simulink model "ASM_Traffic_new"  (R2024a)
settings: Solver=ode1  StartTime=SIM.tstart.v  StopTime=SIM.tend.v  FixedStep=SIM.StepSize.v  RelTol=1e-3
PostLoadFcn:
  | if any(exist('dsrtsu_mdlpostloadfcn', 'file') ~= 0), dsrtsu_mdlpostloadfcn('Execute', bdroot); end
  | try, asm_mdl_postloadfcn(bdroot, 'UpdateModel', 3600); catch, disp(lasterr); end,
InitFcn:
  | , if any(exist('rtifpga_mdlclblib', 'file') ~= 0), rtifpga_mdlclblib('Init', bdroot); end,
  | , if any(exist('dsmpb_private', 'file') ~= 0), dsmpb_private('dsmpb_mdlclblib', 'Init', bdroot); end,
undefined symbols (not defined in the file): _to_, a0b2, ASM_BrakeHydraulics_DemoSystems, ASM_VehicleDynamics_DemoSystems, b98103fe8ad365046cd0, BrakeCircuit, CPT, Crankshaft, DiscIntNeverNeededParam, dsmsi, FinalDriveAssembly, MDL, ModeSignals, Pos_BrakePedal_Maneuver, rad, RefSignals, s_to_rpm, SIM, SoftECU, Suspension, Tire, Transmission
libraries: ASM_Traffic_lib x135, simulink x100, ASM_Utils_lib x77, ASM_VehicleDynamics_lib x70, ASM_Environment_lib x22, dsmpblib x20, dsmsilib x15, MDLD_Utils_lib x10, ASM_BrakeHydraulics_lib x3
(part 18 of 63)

== system ASM_Traffic_new/DomainControl/DriverAssistance/Control/SoftECU_ACC ==
  UserInterface : Inport
  Interface_In : Inport  Port=2
  Bus Creator : BusCreator  Inputs=10
  Bus Selector1 : BusSelector  OutputSignals=SoftECU_ACC.Switches_ACC
  Bus Selector3 : BusSelector  OutputSignals=ExternalModel.v_x_Vehicle_CoG[km|h],ExternalModel.YawRate_Vehicle_CoG[deg|s],ExternalModel.Pos_FL_Wheel[x;y;z][m],ExternalModel.Pos_FR_Wheel[x;y;z][m],ExternalModel.r_Dyn_Tire[FL;FR;RL;RR][m],ExternalModel.Coef_RollingRes[FL;FR;RL;RR][],ExternalModel.Cw_x[],ExternalModel.i_FrontDrive[],ExternalModel.i_RearDrive[],ExternalModel.TrqDistri_Front_Rear[0_1][],ExternalModel.i_unsync_Trm[],ExternalModel.m_TotalVehicle[kg],ExternalModel.Trq_Fric_Engine[Nm],ExternalModel.Pos_AccPedal[%],ExternalModel.Pos_BrakePedal[%],ExternalModel.Slope_Veh_Road[%],ExternalModel.s_Vehicle_Road[m],ExternalModel.d_Vehicle_Road[m],ExternalModel.Dist_Fellows[m],ExternalModel.v_Rel_Fellows[m|s],ExternalModel.Angle_Hor_Rel_Fellows[deg],ExternalModel.s_Fellows_Ref[m],ExternalModel.d_Total_Fellows[m],ExternalModel.PosVec_MainPnt_Fellows[x;y;z][m],ExternalModel.Length_Fellows[m],ExternalModel.Width_Fellows[m],ExternalModel.Height_Fellows[m],ExternalModel.Object_ID[],ExternalModel.ECU_Commands[],ExternalModel.Reset[0|1]
  ModelDesk_MC_ID_SoftECU : ASM_Utils_lib/ModelDeskInterface/ModelDesk_MC  Tag=ASM_MAINCOMPONENT  Editable=off  MainComponent=SoftECU
  Soft_ECU_ACC : Subsystem
  ASMSignalBus : Outport  VectorParamsAs1DForOutWhenUnconnected=off
  Out : Outport  Port=2  VectorParamsAs1DForOutWhenUnconnected=off
  wires:
  Bus Creator/1 -> Out/1
  Soft_ECU_ACC/8(AEB[0|1]) -> Bus Creator/7  "AEB[0|1]"
  Soft_ECU_ACC/7(FCW[0|1]) -> Bus Creator/6  "FCW[0|1]"
  Soft_ECU_ACC/6(Trq_Request_Brake_ACC[Nm]) -> Bus Creator/5  "Trq_DecreaseRequest_ACC[Nm]"
  Soft_ECU_ACC/5(Enable_Trq_Brake_ACC[0|1]) -> Bus Creator/4  "Enable_Trq_Decrease_ACC[0|1]"
  Soft_ECU_ACC/3(Trq_Request_Engine_ACC[Nm]) -> Bus Creator/2  "Trq_IncreaseRequest_ACC[Nm]"
  Soft_ECU_ACC/2(Enable_Trq_Engine_ACC[0|1]) -> Bus Creator/1  "Enable_Trq_Increase_ACC[0|1]"
  Soft_ECU_ACC/1(ASMSignalBus) -> ASMSignalBus/1
  Bus Selector3/30 -> Soft_ECU_ACC/31(Reset[0|1])  "<Reset[0|1]>"
  Bus Selector3/29 -> Soft_ECU_ACC/30(ECU_Commands[])  "<ECU_Commands[]>"
  Bus Selector3/28 -> Soft_ECU_ACC/29(Object_ID[])  "<Object_ID[]>"
  Bus Selector3/27 -> Soft_ECU_ACC/28(Height_Fellows[m])  "<Height_Fellows[m]>"
  Bus Selector3/26 -> Soft_ECU_ACC/27(Width_Fellows[m])  "<Width_Fellows[m]>"
  Bus Selector3/25 -> Soft_ECU_ACC/26(Length_Fellows[m])  "<Length_Fellows[m]>"
  Bus Selector3/24 -> Soft_ECU_ACC/25(PosVec_MainPnt_Fellows[x;y;z][m])  "<PosVec_MainPnt_Fellows[x;y;z][m]>"
  Bus Selector3/23 -> Soft_ECU_ACC/24(d_Total_Fellows[m])  "<d_Total_Fellows[m]>"
  Bus Selector3/22 -> Soft_ECU_ACC/23(s_Fellows_Ref[m])  "<s_Fellows_Ref[m]>"
  Bus Selector3/21 -> Soft_ECU_ACC/22(Angle_Hor_Rel_Fellows[deg])  "<Angle_Hor_Rel_Fellows[deg]>"
  Bus Selector3/20 -> Soft_ECU_ACC/21(v_Rel_Fellows[m|s])  "<v_Rel_Fellows[m|s]>"
  Bus Selector3/19 -> Soft_ECU_ACC/20(Dist_Fellows[m])  "<Dist_Fellows[m]>"
  Bus Selector3/18 -> Soft_ECU_ACC/19(d_Vehicle_Road[m])  "<d_Vehicle_Road[m]>"
  Bus Selector3/17 -> Soft_ECU_ACC/18(s_Vehicle_Road[m])  "<s_Vehicle_Road[m]>"
  Bus Selector3/16 -> Soft_ECU_ACC/17(Slope_Veh_Road[%])  "<Slope_Veh_Road[%]>"
  Bus Selector3/15 -> Soft_ECU_ACC/16(Pos_BrakePedal[%])  "<Pos_BrakePedal[%]>"
  Bus Selector3/14 -> Soft_ECU_ACC/15(Pos_AccPedal[%])  "<Pos_AccPedal[%]>"
  Bus Selector3/13 -> Soft_ECU_ACC/14(Trq_Fric_Engine[Nm])  "<Trq_Fric_Engine[Nm]>"
  Bus Selector3/12 -> Soft_ECU_ACC/13(m_TotalVehicle[kg])  "<m_TotalVehicle[kg]>"
  Bus Selector3/11 -> Soft_ECU_ACC/12(i_unsync_Trm[])  "<i_unsync_Trm[]>"
  Bus Selector3/8 -> Soft_ECU_ACC/9(i_FrontDrive[])  "<i_FrontDrive[]>"
  Bus Selector3/7 -> Soft_ECU_ACC/8(Cw_x[])  "<Cw_x[]>"
  Bus Selector3/6 -> Soft_ECU_ACC/7(Coef_RollingRes[FL;FR;RL;RR][])  "<Coef_RollingRes[FL;FR;RL;RR][]>"
  Bus Selector3/1 -> Soft_ECU_ACC/2(v_x_Vehicle_CoG[km|h])  "<v_x_Vehicle_CoG[km|h]>"
  Bus Selector3/5 -> Soft_ECU_ACC/6(r_Dyn_Tire[FL;FR;RL;RR][m])  "<r_Dyn_Tire[FL;FR;RL;RR][m]>"
  Bus Selector3/2 -> Soft_ECU_ACC/3(YawRate_Vehicle_CoG[deg|s])  "<YawRate_Vehicle_CoG[deg|s]>"
  Bus Selector3/4 -> Soft_ECU_ACC/5(Pos_FR_Wheel[x;y;z][m])  "<Pos_FR_Wheel[x;y;z][m]>"
  Bus Selector3/3 -> Soft_ECU_ACC/4(Pos_FL_Wheel[x;y;z][m])  "<Pos_FL_Wheel[x;y;z][m]>"
  Interface_In/1 -> Bus Selector3/1
  Bus Selector1/1 -> Soft_ECU_ACC/1(Switches_ACC_User)  "<Switches_ACC>"
  UserInterface/1 -> Bus Selector1/1
  Soft_ECU_ACC/4(Trq_Request_Engine_ACC[Front;Rear][Nm]) -> Bus Creator/3  "Trq_IncreaseRequest_ACC[Front;Rear][Nm]"
  Bus Selector3/9 -> Soft_ECU_ACC/10(i_RearDrive[])  "<i_RearDrive[]>"
  Bus Selector3/10 -> Soft_ECU_ACC/11(TrqDistri_Front_Rear[0_1])  "<TrqDistri_Front_Rear[0_1][]>"
  Soft_ECU_ACC/9(ACC_State[1OFF|2Standby|3ON]) -> Bus Creator/8  "ACC_State[1OFF|2Standby|3ON]"
  Soft_ECU_ACC/10(Driver_Override_ACC_Active[0Off|1On]) -> Bus Creator/9  "Driver_Override_ACC_Active[0Off|1On]"
  Soft_ECU_ACC/11(Driver_Override_ACC_Reason[0NoOverride|1BrakePedal|2AccPedal]) -> Bus Creator/10  "Driver_Override_ACC_Reason[0NoOverride|1BrakePedal|2AccPedal]"

== system ASM_Traffic_new/DomainControl/DriverAssistance/Control/Sw_ECU_Signals ==
  SoftECU : Inport
  ExternalECU : Inport  Port=2
  ACC_State[1OFF|2Standby|3ON] : Subsystem
  AEB[0|1] : Subsystem
  Bus Creator1 : BusCreator  Inputs=10
  Bus Selector2 : BusSelector  OutputSignals=Enable_Trq_Increase_ACC[0|1],Trq_IncreaseRequest_ACC[Nm],Trq_IncreaseRequest_ACC[Front;Rear][Nm],Enable_Trq_Decrease_ACC[0|1],Trq_DecreaseRequest_ACC[Nm],FCW[0|1],AEB[0|1],ACC_State[1OFF|2Standby|3ON],Driver_Override_ACC_Active[0Off|1On],Driver_Override_ACC_Reason[0NoOverride|1BrakePedal|2AccPedal]
  Bus Selector3 : BusSelector  OutputSignals=ExternalECU.Enable_Trq_Increase_ACC[0|1],ExternalECU.Trq_IncreaseRequest_ACC[Nm],ExternalECU.Trq_IncreaseRequest_ACC[Front;Rear][Nm],ExternalECU.Enable_Trq_Decrease_ACC[0|1],ExternalECU.Trq_DecreaseRequest_ACC[Nm],ExternalECU.FCW[0|1],ExternalECU.AEB[0|1],ExternalECU.ACC_State[1OFF|2Standby|3ON]
  Enable_Trq_Decrease_ACC[0|1] : Subsystem
  Enable_Trq_Increase_ACC[0|1] : Subsystem
  FCW[0|1] : Subsystem
  Trq_DecreaseRequest_ACC[Nm] : Subsystem
  Trq_IncreaseRequest_ACC[Front;Rear][Nm] : Subsystem
  Trq_IncreaseRequest_ACC[Nm] : Subsystem
  ECU_Signals : Outport  VectorParamsAs1DForOutWhenUnconnected=off
  wires:
  Bus Selector3/7 -> AEB[0|1]/2(RealECU)  "<AEB[0|1]>"
  Bus Selector3/6 -> FCW[0|1]/2(RealECU)  "<FCW[0|1]>"
  AEB[0|1]/1(AEB[0|1]) -> Bus Creator1/7  "AEB[0|1]"
  FCW[0|1]/1(FCW[0|1]) -> Bus Creator1/6  "FCW[0|1]"
  Bus Selector2/7 -> AEB[0|1]/1(SoftECU)  "<AEB[0|1]>"
  Bus Selector2/6 -> FCW[0|1]/1(SoftECU)  "<FCW[0|1]>"
  Bus Selector2/1 -> Enable_Trq_Increase_ACC[0|1]/1(SoftECU)  "<Enable_Trq_Increase_ACC[0|1]>"
  Bus Selector2/5 -> Trq_DecreaseRequest_ACC[Nm]/1(SoftECU)  "<Trq_DecreaseRequest_ACC[Nm]>"
  Bus Selector2/2 -> Trq_IncreaseRequest_ACC[Nm]/1(SoftECU)  "<Trq_IncreaseRequest_ACC[Nm]>"
  Trq_IncreaseRequest_ACC[Nm]/1(Trq_IncreaseRequest_ACC[Nm]) -> Bus Creator1/2  "Trq_IncreaseRequest_ACC[Nm]"
  Bus Selector2/4 -> Enable_Trq_Decrease_ACC[0|1]/1(SoftECU)  "<Enable_Trq_Decrease_ACC[0|1]>"
  Enable_Trq_Increase_ACC[0|1]/1(Enable_Trq_Increase_ACC[0|1]) -> Bus Creator1/1  "Enable_Trq_Increase_ACC[0|1]"
  Enable_Trq_Decrease_ACC[0|1]/1(Enable_Trq_Decrease_ACC[0|1]) -> Bus Creator1/4  "Enable_Trq_Decrease_ACC[0|1]"
  Bus Creator1/1 -> ECU_Signals/1  "ECU_ACC"
  Trq_DecreaseRequest_ACC[Nm]/1(Trq_DecreaseRequest_ACC[Nm]) -> Bus Creator1/5  "Trq_DecreaseRequest_ACC[Nm]"
  ExternalECU/1 -> Bus Selector3/1
  SoftECU/1 -> Bus Selector2/1
  Bus Selector3/1 -> Enable_Trq_Increase_ACC[0|1]/2(RealECU)  "<Enable_Trq_Increase_ACC[0|1]>"
  Bus Selector3/2 -> Trq_IncreaseRequest_ACC[Nm]/2(RealECU)  "<Trq_IncreaseRequest_ACC[Nm]>"
  Bus Selector3/4 -> Enable_Trq_Decrease_ACC[0|1]/2(RealECU)  "<Enable_Trq_Decrease_ACC[0|1]>"
  Bus Selector3/5 -> Trq_DecreaseRequest_ACC[Nm]/2(RealECU)  "<Trq_DecreaseRequest_ACC[Nm]>"
  Bus Selector2/3 -> Trq_IncreaseRequest_ACC[Front;Rear][Nm]/1(SoftECU)  "<Trq_IncreaseRequest_ACC[Front;Rear][Nm]>"
  Trq_IncreaseRequest_ACC[Front;Rear][Nm]/1(Trq_IncreaseRequest_ACC[Front;Rear][Nm]) -> Bus Creator1/3  "Trq_IncreaseRequest_ACC[Front;Rear][Nm]"
  Bus Selector3/3 -> Trq_IncreaseRequest_ACC[Front;Rear][Nm]/2(RealECU)  "<Trq_IncreaseRequest_ACC[Front;Rear][Nm]>"
  Bus Selector2/8 -> ACC_State[1OFF|2Standby|3ON]/1(SoftECU)  "<ACC_State[1OFF|2Standby|3ON]>"
  ACC_State[1OFF|2Standby|3ON]/1(ACC_State[1OFF|2Standby|3ON]) -> Bus Creator1/8  "ACC_State[1OFF|2Standby|3ON]"
  Bus Selector3/8 -> ACC_State[1OFF|2Standby|3ON]/2(RealECU)  "<ACC_State[1OFF|2Standby|3ON]>"
  Bus Selector2/9 -> Bus Creator1/9  "<Driver_Override_ACC_Active[0Off|1On]>"
  Bus Selector2/10 -> Bus Creator1/10  "<Driver_Override_ACC_Reason[0NoOverride|1BrakePedal|2AccPedal]>"

== system ASM_Traffic_new/DomainControl/DriverAssistance/Control/UserInterface ==
  note: Driver Assistance
  Interface_In : Inport
  In : Inport  Port=2
  ASMSignalBus_Control : Subsystem
  DISP_Control : Subsystem
  PAR_Control : Subsystem
  Out : Outport  VectorParamsAs1DForOutWhenUnconnected=off
  wires:
  Interface_In/1 -> DISP_Control/1(Interface_In)
  In/1 -> ASMSignalBus_Control/1(In), DISP_Control/2(In)
  PAR_Control/1(Out) -> Out/1

== system ASM_Traffic_new/DomainControl/DriverAssistance/Interface_In/ExternalSignals ==
  Enable : EnablePort
  ExternalECU_ACC : Subsystem
  ExternalECU_ACC_In : dsmpblib/Data Inport  Tag=ASM_MPB  Priority=10000
      settings: SourceProductName=dSPACE Model Interface Package for Simulink (MIPS)
  ExternalECU_ACC_Out : Outport
  wires:
  ExternalECU_ACC/1(Out) -> ExternalECU_ACC_Out/1
  ExternalECU_ACC_In/8 -> ExternalECU_ACC/8(ACC_State[1OFF|2Standby|3ON])
  ExternalECU_ACC_In/7 -> ExternalECU_ACC/7(AEB[0|1])
  ExternalECU_ACC_In/6 -> ExternalECU_ACC/6(FCW[0|1])
  ExternalECU_ACC_In/5 -> ExternalECU_ACC/5(Trq_DecreaseRequest_ACC[Nm])
  ExternalECU_ACC_In/4 -> ExternalECU_ACC/4(Enable_Trq_Decrease_ACC[0|1])
  ExternalECU_ACC_In/3 -> ExternalECU_ACC/3(Trq_IncreaseRequest_ACC[Front;Rear][Nm])
  ExternalECU_ACC_In/2 -> ExternalECU_ACC/2(Trq_IncreaseRequest_ACC[Nm])
  ExternalECU_ACC_In/1 -> ExternalECU_ACC/1(Enable_Trq_Increase_ACC[0|1])

== system ASM_Traffic_new/DomainControl/DriverAssistance/Interface_In/ModelSignals ==
  Sw_ModelPortBlocks[0Disabled|1Enabled] : Inport
  Sw_ModelDeskPlottingInterface[0Disabled|1Enabled] : Inport  Port=2
  v_x_Vehicle_CoG[km|h] : Inport  Port=3
  YawRate_Vehicle_CoG[deg|s] : Inport  Port=4
  Pos_FL_Wheel[x;y;z][m] : Inport  Port=5
  Pos_FR_Wheel[x;y;z][m] : Inport  Port=6
  r_Dyn_Tire[FL;FR;RL;RR][m] : Inport  Port=7
  Coef_RollingRes[FL;FR;RL;RR][] : Inport  Port=8
  Cw_x[] : Inport  Port=9
  m_TotalVehicle[kg] : Inport  Port=10
  i_FrontDrive[] : Inport  Port=11
  i_RearDrive[] : Inport  Port=12
  TrqDistri_Front_Rear[0_1][] : Inport  Port=13
  i_unsync_Trm[] : Inport  Port=14
  Pos_AccPedal[%] : Inport  Port=15
  Pos_BrakePedal[%] : Inport  Port=16
  Slope_Veh_Road[%] : Inport  Port=17
  s_Vehicle_Road[m] : Inport  Port=18
  d_Vehicle_Road[m] : Inport  Port=19
  ECU_Commands[] : Inport  Port=20
  Reset[0|1] : Inport  Port=21
  Dist_Fellows[m] : Inport  Port=22
  v_Rel_Fellows[m|s] : Inport  Port=23
  Angle_Hor_Rel_Fellows[deg] : Inport  Port=24
  s_Fellows_Ref[m] : Inport  Port=25
  d_Total_Fellows[m] : Inport  Port=26
  PosVec_MainPnt_Fellows[x;y;z][m] : Inport  Port=27
  Length_Fellows[m] : Inport  Port=28
  Width_Fellows[m] : Inport  Port=29
  Height_Fellows[m] : Inport  Port=30
  Object_ID[] : Inport  Port=31
  v_Vehicle[km|h] : Inport  Port=32
  Trq_Fric_Engine[Nm] : Inport  Port=33
  Angle_Hor_Rel_Fellows[deg]_ : Subsystem
      mask Display: disp('')
  Bus Creator1 : BusCreator  Inputs=33
  Coef_RollingRes[FL;FR;RL;RR][]_ : Subsystem
      mask Display: disp('')
  Cw_x[]_ : Subsystem
      mask Display: disp('')
  Dist_Fellows[m]_ : Subsystem
      mask Display: disp('')
  ECU_Commands[]_ : Subsystem
      mask Display: disp('')
  Height_Fellows[m]_ : Subsystem
      mask Display: disp('')
  Length_Fellows[m]_ : Subsystem
      mask Display: disp('')
  Object_ID[]_ : Subsystem
      mask Display: disp('')
  PosVec_MainPnt_Fellows[x;y;z][m]_ : Subsystem
      mask Display: disp('')
  Pos_AccPedal[%]_ : Subsystem
      mask Display: disp('')
  Pos_BrakePedal[%]_ : Subsystem
      mask Display: disp('')
  Pos_FL_Wheel[x;y;z][m]_ : Subsystem
      mask Display: disp('')
  Pos_FR_Wheel[x;y;z][m]_ : Subsystem
      mask Display: disp('')
  Reset[0|1]_ : Subsystem
      mask Display: disp('')
  Slope_Veh_Road[%]_ : Subsystem
      mask Display: disp('')
  Sw_ModelDeskPlottingInterface[0Disabled|1Enabled]_ : Subsystem
  Sw_ModelPortBlocks[0Disabled|1Enabled]_ : Subsystem
  TrqDistri_Front_Rear[0_1][]_ : Subsystem
      mask Display: disp('')
  Trq_Fric_Engine[Nm]_ : Subsystem
      mask Display: disp('')
  Width_Fellows[m]_ : Subsystem
      mask Display: disp('')
  YawRate_Vehicle_CoG[deg|s]_ : Subsystem
      mask Display: disp('')
  d_Total_Fellows[m]_ : Subsystem
      mask Display: disp('')
  d_Vehicle_Road[m]_ : Subsystem
      mask Display: disp('')
  i_FrontDrive[]_ : Subsystem
      mask Display: disp('')
  i_RearDrive[]_ : Subsystem
      mask Display: disp('')
  i_unsync_Trm[]_ : Subsystem
      mask Display: disp('')
  m_TotalVehicle[kg]_ : Subsystem
      mask Display: disp('')
  r_Dyn_Tire[FL;FR;RL;RR][m]_ : Subsystem
      mask Display: disp('')
  s_Fellows_Ref[m]_ : Subsystem
      mask Display: disp('')
  s_Vehicle_Road[m]_ : Subsystem
      mask Display: disp('')
  v_Rel_Fellows[m|s]_ : Subsystem
      mask Display: disp('')
  v_Vehicle[km|h]_ : Subsystem
      mask Display: disp('')
  v_x_Vehicle_CoG[km|h]_ : Subsystem
      mask Display: disp('')
  Out : Outport  VectorParamsAs1DForOutWhenUnconnected=off
  wires:
  Sw_ModelDeskPlottingInterface[0Disabled|1Enabled]_/1(Out1) -> Bus Creator1/2  "Sw_ModelDeskPlottingInterface[0Disabled|1Enabled]"
  Sw_ModelPortBlocks[0Disabled|1Enabled]_/1(Out1) -> Bus Creator1/1  "Sw_ModelPortBlocks[0Disabled|1Enabled]"
  Sw_ModelDeskPlottingInterface[0Disabled|1Enabled]/1 -> Sw_ModelDeskPlottingInterface[0Disabled|1Enabled]_/1(In1)
  Sw_ModelPortBlocks[0Disabled|1Enabled]/1 -> Sw_ModelPortBlocks[0Disabled|1Enabled]_/1(In1)
  Bus Creator1/1 -> Out/1  "ExternalModel"
  v_Vehicle[km|h]_/1(Out1) -> Bus Creator1/32  "v_Vehicle[km|h]"
  v_Vehicle[km|h]/1 -> v_Vehicle[km|h]_/1(In1)
  Reset[0|1]_/1(Out1) -> Bus Creator1/31  "Reset[0|1]"
  ECU_Commands[]_/1(Out1) -> Bus Creator1/30  "ECU_Commands[]"
  Object_ID[]_/1(Out1) -> Bus Creator1/29  "Object_ID[]"
  Height_Fellows[m]_/1(Out1) -> Bus Creator1/28  "Height_Fellows[m]"
  Width_Fellows[m]_/1(Out1) -> Bus Creator1/27  "Width_Fellows[m]"
  Length_Fellows[m]_/1(Out1) -> Bus Creator1/26  "Length_Fellows[m]"
  PosVec_MainPnt_Fellows[x;y;z][m]_/1(Out1) -> Bus Creator1/25  "PosVec_MainPnt_Fellows[x;y;z][m]"
  d_Total_Fellows[m]_/1(Out1) -> Bus Creator1/24  "d_Total_Fellows[m]"
  s_Fellows_Ref[m]_/1(Out1) -> Bus Creator1/23  "s_Fellows_Ref[m]"
  Angle_Hor_Rel_Fellows[deg]_/1(Out1) -> Bus Creator1/22  "Angle_Hor_Rel_Fellows[deg]"
  v_Rel_Fellows[m|s]_/1(Out1) -> Bus Creator1/21  "v_Rel_Fellows[m|s]"
  Dist_Fellows[m]_/1(Out1) -> Bus Creator1/20  "Dist_Fellows[m]"
  d_Vehicle_Road[m]_/1(Out1) -> Bus Creator1/19  "d_Vehicle_Road[m]"
  s_Vehicle_Road[m]_/1(Out1) -> Bus Creator1/18  "s_Vehicle_Road[m]"
  Slope_Veh_Road[%]_/1(Out1) -> Bus Creator1/17  "Slope_Veh_Road[%]"
  Pos_BrakePedal[%]_/1(Out1) -> Bus Creator1/16  "Pos_BrakePedal[%]"
  Pos_AccPedal[%]_/1(Out1) -> Bus Creator1/15  "Pos_AccPedal[%]"
  Trq_Fric_Engine[Nm]_/1(Out1) -> Bus Creator1/33  "Trq_Fric_Engine[Nm]"
  TrqDistri_Front_Rear[0_1][]_/1(Out1) -> Bus Creator1/13  "TrqDistri_Front_Rear[0_1][]"
  Cw_x[]_/1(Out1) -> Bus Creator1/9  "Cw_x[]"
  Coef_RollingRes[FL;FR;RL;RR][]_/1(Out1) -> Bus Creator1/8  "Coef_RollingRes[FL;FR;RL;RR][]"
  r_Dyn_Tire[FL;FR;RL;RR][m]_/1(Out1) -> Bus Creator1/7  "r_Dyn_Tire[FL;FR;RL;RR][m]"
  Pos_FR_Wheel[x;y;z][m]_/1(Out1) -> Bus Creator1/6  "Pos_FR_Wheel[x;y;z][m]"
  Pos_FL_Wheel[x;y;z][m]_/1(Out1) -> Bus Creator1/5  "Pos_FL_Wheel[x;y;z][m]"
  YawRate_Vehicle_CoG[deg|s]_/1(Out1) -> Bus Creator1/4  "YawRate_Vehicle_CoG[deg|s]"
  v_x_Vehicle_CoG[km|h]_/1(Out1) -> Bus Creator1/3  "v_x_Vehicle_CoG[km|h]"
  Reset[0|1]/1 -> Reset[0|1]_/1(In1)
  ECU_Commands[]/1 -> ECU_Commands[]_/1(In1)
  Object_ID[]/1 -> Object_ID[]_/1(In1)
  Height_Fellows[m]/1 -> Height_Fellows[m]_/1(In1)
  Width_Fellows[m]/1 -> Width_Fellows[m]_/1(In1)
  Length_Fellows[m]/1 -> Length_Fellows[m]_/1(In1)
  PosVec_MainPnt_Fellows[x;y;z][m]/1 -> PosVec_MainPnt_Fellows[x;y;z][m]_/1(In1)
  d_Total_Fellows[m]/1 -> d_Total_Fellows[m]_/1(In1)
  s_Fellows_Ref[m]/1 -> s_Fellows_Ref[m]_/1(In1)
  Angle_Hor_Rel_Fellows[deg]/1 -> Angle_Hor_Rel_Fellows[deg]_/1(In1)
  v_Rel_Fellows[m|s]/1 -> v_Rel_Fellows[m|s]_/1(In1)
  Dist_Fellows[m]/1 -> Dist_Fellows[m]_/1(In1)
  d_Vehicle_Road[m]/1 -> d_Vehicle_Road[m]_/1(In1)
  s_Vehicle_Road[m]/1 -> s_Vehicle_Road[m]_/1(In1)
  Slope_Veh_Road[%]/1 -> Slope_Veh_Road[%]_/1(In1)
  Pos_BrakePedal[%]/1 -> Pos_BrakePedal[%]_/1(In1)
  Pos_AccPedal[%]/1 -> Pos_AccPedal[%]_/1(In1)
  Trq_Fric_Engine[Nm]/1 -> Trq_Fric_Engine[Nm]_/1(In1)
  m_TotalVehicle[kg]/1 -> m_TotalVehicle[kg]_/1(In1)
  i_FrontDrive[]/1 -> i_FrontDrive[]_/1(In1)
  Cw_x[]/1 -> Cw_x[]_/1(In1)
  Coef_RollingRes[FL;FR;RL;RR][]/1 -> Coef_RollingRes[FL;FR;RL;RR][]_/1(In1)
  r_Dyn_Tire[FL;FR;RL;RR][m]/1 -> r_Dyn_Tire[FL;FR;RL;RR][m]_/1(In1)
  Pos_FR_Wheel[x;y;z][m]/1 -> Pos_FR_Wheel[x;y;z][m]_/1(In1)
  Pos_FL_Wheel[x;y;z][m]/1 -> Pos_FL_Wheel[x;y;z][m]_/1(In1)
  YawRate_Vehicle_CoG[deg|s]/1 -> YawRate_Vehicle_CoG[deg|s]_/1(In1)
  v_x_Vehicle_CoG[km|h]/1 -> v_x_Vehicle_CoG[km|h]_/1(In1)
  i_unsync_Trm[]/1 -> i_unsync_Trm[]_/1(In1)
  i_unsync_Trm[]_/1(Out1) -> Bus Creator1/14  "i_unsync_Trm[]"
  i_RearDrive[]/1 -> i_RearDrive[]_/1(In1)
  TrqDistri_Front_Rear[0_1][]/1 -> TrqDistri_Front_Rear[0_1][]_/1(In1)
  m_TotalVehicle[kg]_/1(Out1) -> Bus Creator1/10  "m_TotalVehicle[kg]"
  i_FrontDrive[]_/1(Out1) -> Bus Creator1/11  "i_FrontDrive[]"
  i_RearDrive[]_/1(Out1) -> Bus Creator1/12  "i_RearDrive[]"

== system ASM_Traffic_new/DomainControl/DriverAssistance/Interface_Out/Animation ==
  State_ACC[0Off|1On] : Inport
  Target_Detected[0|1] : Inport  Port=2
  v_Set[km|h] : Inport  Port=3
  Distance_Set[m] : Inport  Port=4
  Dist_Long[m] : Inport  Port=5
  BusCreator1 : BusCreator  Inputs=5
  Dist_Long[m]_ : Subsystem
      mask Display: disp('')
  Distance_Set[m]_ : Subsystem
      mask Display: disp('')
  State_ACC[0Off|1On]_ : Subsystem
      mask Display: disp('')
  Target_Detected[0|1]_ : Subsystem
      mask Display: disp('')
  v_Set[km|h]_ : Subsystem
      mask Display: disp('')
  Out : Outport  VectorParamsAs1DForOutWhenUnconnected=off
  wires:
  BusCreator1/1 -> Out/1  "Animation"
  Dist_Long[m]_/1(Out1) -> BusCreator1/5  "Dist_Long[m]"
  Distance_Set[m]_/1(Out1) -> BusCreator1/4  "Distance_Set[m]"
  v_Set[km|h]_/1(Out1) -> BusCreator1/3  "v_Set[km|h]"
  Target_Detected[0|1]_/1(Out1) -> BusCreator1/2  "Target_Detected[0|1]"
  State_ACC[0Off|1On]_/1(Out1) -> BusCreator1/1  "State_ACC[0Off|1On]"
  v_Set[km|h]/1 -> v_Set[km|h]_/1(In1)
  Dist_Long[m]/1 -> Dist_Long[m]_/1(In1)
  Distance_Set[m]/1 -> Distance_Set[m]_/1(In1)
  Target_Detected[0|1]/1 -> Target_Detected[0|1]_/1(In1)
  State_ACC[0Off|1On]/1 -> State_ACC[0Off|1On]_/1(In1)

== system ASM_Traffic_new/DomainControl/DriverAssistance/Interface_Out/Control_ModelSignals ==
  Enable_Trq_Increase_ACC[0|1] : Inport
  Trq_IncreaseRequest_ACC[Nm] : Inport  Port=2
  Trq_IncreaseRequest_ACC[Front;Rear][Nm] : Inport  Port=3
  Enable_Trq_Decrease_ACC[0|1] : Inport  Port=4
  Trq_DecreaseRequest_ACC[Nm] : Inport  Port=5
  AEB[0|1] : Inport  Port=6
  FCW[0|1] : Inport  Port=7
  ACC_State[1OFF|2Standby|3ON] : Inport  Port=8
  Driver_Override_ACC_Active[0Off|1On] : Inport  Port=9
  Driver_Override_ACC_Reason[0NoOverride|1BrakePedal|2AccPedal] : Inport  Port=10
  ACC_State[1OFF|2Standby|3ON]_ : Subsystem
      mask Display: disp('')
  AEB[0|1]_ : Subsystem
      mask Display: disp('')
  Bus Creator : BusCreator  Inputs=10
  Driver_Override_ACC_Active[0Off|1On]_ : Subsystem
      mask Display: disp('')
  Driver_Override_ACC_Reason[0NoOverride|1BrakePedal|2AccPedal]_ : Subsystem
      mask Display: disp('')
  Enable_Trq_Decrease_ACC[0|1]_ : Subsystem
      mask Display: disp('')
  Enable_Trq_Increase_ACC[0|1]_ : Subsystem
      mask Display: disp('')
  FCW[0|1]_ : Subsystem
      mask Display: disp('')
  Trq_DecreaseRequest_ACC[Nm]_ : Subsystem
      mask Display: disp('')
  Trq_IncreaseRequest_ACC[Front;Rear][Nm]_ : Subsystem
      mask Display: disp('')
  Trq_IncreaseRequest_ACC[Nm]_ : Subsystem
      mask Display: disp('')
  Out : Outport  VectorParamsAs1DForOutWhenUnconnected=off
  wires:
  Trq_DecreaseRequest_ACC[Nm]/1 -> Trq_DecreaseRequest_ACC[Nm]_/1(In1)
  Enable_Trq_Decrease_ACC[0|1]/1 -> Enable_Trq_Decrease_ACC[0|1]_/1(In1)
  Enable_Trq_Decrease_ACC[0|1]_/1(Out1) -> Bus Creator/4  "Enable_Trq_Decrease_ACC[0|1]"
  Trq_DecreaseRequest_ACC[Nm]_/1(Out1) -> Bus Creator/5  "Trq_DecreaseRequest_ACC[Nm]"
  Bus Creator/1 -> Out/1  "Control"
  Trq_IncreaseRequest_ACC[Nm]_/1(Out1) -> Bus Creator/2  "Trq_IncreaseRequest_ACC[Nm]"
  Enable_Trq_Increase_ACC[0|1]_/1(Out1) -> Bus Creator/1  "Enable_Trq_Increase_ACC[0|1]"
  Enable_Trq_Increase_ACC[0|1]/1 -> Enable_Trq_Increase_ACC[0|1]_/1(In1)
  Trq_IncreaseRequest_ACC[Nm]/1 -> Trq_IncreaseRequest_ACC[Nm]_/1(In1)
  Trq_IncreaseRequest_ACC[Front;Rear][Nm]/1 -> Trq_IncreaseRequest_ACC[Front;Rear][Nm]_/1(In1)
  Trq_IncreaseRequest_ACC[Front;Rear][Nm]_/1(Out1) -> Bus Creator/3  "Trq_IncreaseRequest_ACC[Front;Rear][Nm]"
  AEB[0|1]_/1(Out1) -> Bus Creator/6  "AEB[0|1]"
  FCW[0|1]_/1(Out1) -> Bus Creator/7  "FCW[0|1]"
  AEB[0|1]/1 -> AEB[0|1]_/1(In1)
  FCW[0|1]/1 -> FCW[0|1]_/1(In1)
  ACC_State[1OFF|2Standby|3ON]/1 -> ACC_State[1OFF|2Standby|3ON]_/1(In1)
  ACC_State[1OFF|2Standby|3ON]_/1(Out1) -> Bus Creator/8  "ACC_State[1OFF|2Standby|3ON]"
  Driver_Override_ACC_Active[0Off|1On]_/1(Out1) -> Bus Creator/9  "Driver_Override_ACC_Active[0Off|1On]"
  Driver_Override_ACC_Active[0Off|1On]/1 -> Driver_Override_ACC_Active[0Off|1On]_/1(In1)
  Driver_Override_ACC_Reason[0NoOverride|1BrakePedal|2AccPedal]/1 -> Driver_Override_ACC_Reason[0NoOverride|1BrakePedal|2AccPedal]_/1(In1)
  Driver_Override_ACC_Reason[0NoOverride|1BrakePedal|2AccPedal]_/1(Out1) -> Bus Creator/10  "Driver_Override_ACC_Reason[0NoOverride|1BrakePedal|2AccPedal]"

== system ASM_Traffic_new/DomainControl/DriverAssistance/SignalInterface/ASMSignalInterface ==
  ASMSignalBus : Inport
  Enable : EnablePort
  signal_structure : Subsystem
  wires:
  ASMSignalBus/1 -> signal_structure/1(ASMSignalBus)

== system ASM_Traffic_new/DomainControl/DriverAssistance/SignalInterface/ExternalOutports ==
  In1 : Inport
  Enable : EnablePort
  DriverAssistance : dsmpblib/Data Outport  Tag=ASM_MPB  Priority=-10000
      settings: SourceProductName=dSPACE Model Interface Package for Simulink (MIPS)
  Select_Outport_Signals : Subsystem
  wires:
  In1/1 -> Select_Outport_Signals/1(ASMSignalBus)
  Select_Outport_Signals/4(Target_Selection_ACC) -> DriverAssistance/4
  Select_Outport_Signals/3(Operator_Interface_ACC) -> DriverAssistance/3
  Select_Outport_Signals/2(Interface_ACC) -> DriverAssistance/2
  Select_Outport_Signals/1(Controller_ACC) -> DriverAssistance/1

== system ASM_Traffic_new/DomainControl/StartSystem/Control/SoftECU_StartSystem ==
  note: -------------
  note: Plant
  note: -------------
  note: User Interface
  note: Control
  note: -------------
  note: Inport colors:
  note: External Signals
  note: -------------
  UserInterface : Inport
  Interface_In : Inport  Port=2
  ASMBUS_ENGINE : GotoTagVisibility  GotoTag=ASMBUS_START_BUTTON
  ASMSignalCollector : Subsystem
  Bus Creator5 : BusCreator  Inputs=3
  Bus Selector1 : BusSelector  OutputSignals=ExternalModel.State_StartButton[-1PowerOff|0Acc|1PowerOn|2StarterOn],ExternalModel.Mode_StartButtonState[1Stim|2SoftECU],ExternalModel.Sw_StartButton[0Off|1On],ExternalModel.SelectorLever[-3T|-2P|-1R|0N|1D],ExternalModel.Pos_BrakePedal[%],ExternalModel.Pos_ClutchPedal[%],ExternalModel.State_Engine[0|1|2|3|4],ExternalModel.Reset_States[0|1],ExternalModel.Sw_CrankShaft_Reset[0Disabled|1Enabled]
  Bus Selector2 : BusSelector  OutputSignals=ExternalModel.Mode_Transmission[1Manual|2Automatic]
  Bus Selector4 : BusSelector  OutputSignals=State_KeyFob[1NotAuthorized|2Authorized]
  DisableReset : Subsystem
      mask Display: disp('DisableReset')
  ModelDesk_MC_ID_SoftECU : ASM_Utils_lib/ModelDeskInterface/ModelDesk_MC  Tag=ASM_MAINCOMPONENT  Editable=off  MainComponent=SoftECU
  START_BUTTON : ASM_VehicleDynamics_lib/SoftECU/SoftECU_Body/START_BUTTON  Tag=ASM_SUBCOMPONENT  Const_t_Min_Active=MDL.SoftECU.StartButton.Const_t_Min_Active  Const_t_Min_Starter=MDL.SoftECU.StartButton.Const_t_Min_Starter  Const_Post_ClutchPedal_LowLim=MDL.SoftECU.StartButton.Const_Post_ClutchPedal_LowLim  Const_Post_BrakePedal_LowLim=MDL.SoftECU.StartButton.Const_Post_BrakePedal_LowLim  StepSize=SIM.StepSize  ASMProperties=struct('Name','START_BUTTON','Version','2.0','Library','ASM_VehicleDynamics_lib')  ASMInstanceName=start_button  ASMInstanceID=1
  Terminator_3 : Terminator
  Terminator_4 : Terminator
  ASMSignalBus : Outport  VectorParamsAs1DForOutWhenUnconnected=off
  Out : Outport  Port=2  VectorParamsAs1DForOutWhenUnconnected=off
  tag scope: ASMBUS_START_BUTTON=scoped
  wires:
  START_BUTTON/1 -> [ASMBUS_START_BUTTON]
  ASMSignalCollector/1(ASMSIgnalBus) -> ASMSignalBus/1
  Interface_In/1 -> Bus Selector1/1, Bus Selector2/1
  DisableReset/1(Reset[0|1]) -> START_BUTTON/10
  Bus Selector1/2 -> START_BUTTON/4  "<Mode_StartButtonState[1Stim|2SoftECU]>"
  START_BUTTON/6 -> Bus Creator5/3  "Sw_StarterReq[0|1]"
  START_BUTTON/5 -> Bus Creator5/2  "Sw_Ignition[0|1]"
  Bus Creator5/1 -> Out/1  "ECU_StartSystem"
  Bus Selector1/3 -> START_BUTTON/5  "<Sw_StartButton[0Off|1On]>"
  Bus Selector1/4 -> START_BUTTON/6  "<SelectorLever[-3T|-2P|-1R|0N|1D]>"
  Bus Selector1/5 -> START_BUTTON/7  "<Pos_BrakePedal[%]>"
  Bus Selector1/6 -> START_BUTTON/8  "<Pos_ClutchPedal[%]>"
  Bus Selector1/7 -> START_BUTTON/9  "<State_Engine[0|1|2|3|4]>"
  Bus Selector1/8 -> DisableReset/1(Reset_VehicleStates[0|1])  "<Reset_States[0|1]>"
  Bus Selector1/9 -> DisableReset/2(Sw_CrankShaft_Reset[0Disabled|1Enabled])  "<Sw_CrankShaft_Reset[0Disabled|1Enabled]>"
  UserInterface/1 -> Bus Selector4/1
  Bus Selector4/1 -> START_BUTTON/2  "<State_KeyFob[1NotAuthorized|2Authorized]>"
  START_BUTTON/2 -> Bus Creator5/1  "State_StartButton[-2|-1|0|1|2|3]"
  START_BUTTON/3 -> Terminator_3/1
  START_BUTTON/4 -> Terminator_4/1
  Bus Selector1/1 -> START_BUTTON/3  "<State_StartButton[-1PowerOff|0Acc|1PowerOn|2StarterOn]>"
  Bus Selector2/1 -> START_BUTTON/1  "<Mode_Transmission[1Manual|2Automatic]>"

== system ASM_Traffic_new/DomainControl/StartSystem/Control/Sw_ECU_Signals ==
  SoftECU : Inport
  ExternalECU : Inport  Port=2
  Bus Creator4 : BusCreator  Inputs=3
  Bus Selector1 : BusSelector  OutputSignals=ExternalECU.State_StartButton[-2|-1|0|1|2|3],ExternalECU.Sw_Ignition[0|1],ExternalECU.Sw_StarterReq[0|1]
  Bus Selector2 : BusSelector  OutputSignals=State_StartButton[-2|-1|0|1|2|3],Sw_Ignition[0|1],Sw_StarterReq[0|1]
  State_StartButton[-2|-1|0|1|2|3] : Subsystem
  Sw_Ignition[0|1] : Subsystem
  Sw_StarterReq[0|1] : Subsystem
  ECU_Signals : Outport  VectorParamsAs1DForOutWhenUnconnected=off
  wires:
  Bus Creator4/1 -> ECU_Signals/1  "Control"
  SoftECU/1 -> Bus Selector2/1
  ExternalECU/1 -> Bus Selector1/1
  Bus Selector2/3 -> Sw_StarterReq[0|1]/1(SoftECU)  "<Sw_StarterReq[0|1]>"
  Sw_Ignition[0|1]/1(Sw_Ignition[0|1]) -> Bus Creator4/2  "Sw_Ignition[0|1]"
  Sw_StarterReq[0|1]/1(Sw_StarterReq[0|1]) -> Bus Creator4/3  "Sw_StarterReq[0|1]"
  Bus Selector2/2 -> Sw_Ignition[0|1]/1(SoftECU)  "<Sw_Ignition[0|1]>"
  Bus Selector1/2 -> Sw_Ignition[0|1]/2(RealECU)  "<Sw_Ignition[0|1]>"
  Bus Selector1/3 -> Sw_StarterReq[0|1]/2(RealECU)  "<Sw_StarterReq[0|1]>"
  Bus Selector1/1 -> State_StartButton[-2|-1|0|1|2|3]/2(RealECU)  "<State_StartButton[-2|-1|0|1|2|3]>"
  Bus Selector2/1 -> State_StartButton[-2|-1|0|1|2|3]/1(SoftECU)  "<State_StartButton[-2|-1|0|1|2|3]>"
  State_StartButton[-2|-1|0|1|2|3]/1(State_StartButton[-2|-1|0|1|2|3]) -> Bus Creator4/1  "State_StartButton[-2|-1|0|1|2|3]"

== system ASM_Traffic_new/DomainControl/StartSystem/Control/UserInterface ==
  note: Start System
  Interface_In : Inport
  In : Inport  Port=2
  ASMSignalBus_Control : Subsystem
  DISP_Control : Subsystem
  PAR_Control : Subsystem
  Out : Outport  VectorParamsAs1DForOutWhenUnconnected=off
  wires:
  Interface_In/1 -> DISP_Control/2(Interface_In)
  PAR_Control/1(Out) -> Out/1
  In/1 -> DISP_Control/1(In), ASMSignalBus_Control/1(In)

== system ASM_Traffic_new/DomainControl/StartSystem/Interface_In/ExternalSignals ==
  Enable : EnablePort
  ExternalECU_StartSystem : Subsystem
  ExternalECU_StartSystem_In : dsmpblib/Data Inport  Tag=ASM_MPB  Priority=10000
      settings: SourceProductName=dSPACE Model Interface Package for Simulink (MIPS)
  ExternalECU_StartSystem_Out : Outport
  wires:
  ExternalECU_StartSystem/1(Out) -> ExternalECU_StartSystem_Out/1
  ExternalECU_StartSystem_In/3 -> ExternalECU_StartSystem/3(Sw_StarterReq[0|1])
  ExternalECU_StartSystem_In/2 -> ExternalECU_StartSystem/2(Sw_Ignition[0|1])
  ExternalECU_StartSystem_In/1 -> ExternalECU_StartSystem/1(State_StartButton[-2|-1|0|1|2|3])

== system ASM_Traffic_new/DomainControl/StartSystem/Interface_In/ModelSignals ==
  Sw_ModelPortBlocks[0Disabled|1Enabled] : Inport
  Sw_ModelDeskPlottingInterface[0Disabled|1Enabled] : Inport  Port=2
  Pos_BrakePedal[%] : Inport  Port=3
  Pos_ClutchPedal[%] : Inport  Port=4
  SelectorLever[-3T|-2P|-1R|0N|1D] : Inport  Port=5  PortDimensions=1
  Reset_States[0|1] : Inport  Port=6
  Sw_StartButton[0Off|1On] : Inport  Port=7
  State_Engine[0|1|2|3|4] : Inport  Port=8
  State_StartButton[-1PowerOff|0Acc|1PowerOn|2StarterOn] : Inport  Port=9
  Mode_Transmission[1Manual|2Automatic] : Inport  Port=10
  Sw_CrankShaft_Reset[0Disabled|1Enabled] : Inport  Port=11
  Mode_StartButtonState[1Stim|2SoftECU] : Inport  Port=12
  Bus Creator : BusCreator  Inputs=12
  Mode_StartButtonState[1Stim|2SoftECU]_ : Subsystem
      mask Display: disp('')
  Mode_Transmission[1Manual|2Automatic]_ : Subsystem
      mask Display: disp('')
  Pos_BrakePedal[%]_ : Subsystem
      mask Display: disp('')
  Pos_ClutchPedal[%]_ : Subsystem
      mask Display: disp('')
  Reset_States[0|1]_ : Subsystem
      mask Display: disp('')
  SelectorLever[-3T|-2P|-1R|0N|1D]_ : Subsystem
      mask Display: disp('')
  State_Engine[0|1|2|3|4]_ : Subsystem
      mask Display: disp('')
  State_StartButton[-1PowerOff|0Acc|1PowerOn|2StarterOn]_ : Subsystem
      mask Display: disp('')
  Sw_CrankShaft_Reset[0Disabled|1Enabled]_ : Subsystem
      mask Display: disp('')
  Sw_ModelDeskPlottingInterface[0Disabled|1Enabled]_ : Subsystem
  Sw_ModelPortBlocks[0Disabled|1Enabled]_ : Subsystem
  Sw_StartButton[0Off|1On]_ : Subsystem
      mask Display: disp('')
  Out : Outport  VectorParamsAs1DForOutWhenUnconnected=off
  wires:
  Sw_ModelDeskPlottingInterface[0Disabled|1Enabled]_/1(Out1) -> Bus Creator/2  "Sw_ModelDeskPlottingInterface[0Disabled|1Enabled]"
  Sw_ModelPortBlocks[0Disabled|1Enabled]_/1(Out1) -> Bus Creator/1  "Sw_ModelPortBlocks[0Disabled|1Enabled]"
  Sw_ModelDeskPlottingInterface[0Disabled|1Enabled]/1 -> Sw_ModelDeskPlottingInterface[0Disabled|1Enabled]_/1(In1)
  Sw_ModelPortBlocks[0Disabled|1Enabled]/1 -> Sw_ModelPortBlocks[0Disabled|1Enabled]_/1(In1)
  Bus Creator/1 -> Out/1  "ExternalModel"
  State_Engine[0|1|2|3|4]_/1(Out1) -> Bus Creator/8  "State_Engine[0|1|2|3|4]"
  State_Engine[0|1|2|3|4]/1 -> State_Engine[0|1|2|3|4]_/1(In1)
  Reset_States[0|1]_/1(Out1) -> Bus Creator/6  "Reset_States[0|1]"
  SelectorLever[-3T|-2P|-1R|0N|1D]_/1(Out1) -> Bus Creator/5  "SelectorLever[-3T|-2P|-1R|0N|1D]"
  Sw_StartButton[0Off|1On]_/1(Out1) -> Bus Creator/7  "Sw_StartButton[0Off|1On]"
  Pos_ClutchPedal[%]_/1(Out1) -> Bus Creator/4  "Pos_ClutchPedal[%]"
  Pos_BrakePedal[%]_/1(Out1) -> Bus Creator/3  "Pos_BrakePedal[%]"
  Sw_StartButton[0Off|1On]/1 -> Sw_StartButton[0Off|1On]_/1(In1)
  Pos_BrakePedal[%]/1 -> Pos_BrakePedal[%]_/1(In1)
  Pos_ClutchPedal[%]/1 -> Pos_ClutchPedal[%]_/1(In1)
  SelectorLever[-3T|-2P|-1R|0N|1D]/1 -> SelectorLever[-3T|-2P|-1R|0N|1D]_/1(In1)
  Reset_States[0|1]/1 -> Reset_States[0|1]_/1(In1)
  State_StartButton[-1PowerOff|0Acc|1PowerOn|2StarterOn]_/1(Out1) -> Bus Creator/9  "State_StartButton[-1PowerOff|0Acc|1PowerOn|2StarterOn]"
  State_StartButton[-1PowerOff|0Acc|1PowerOn|2StarterOn]/1 -> State_StartButton[-1PowerOff|0Acc|1PowerOn|2StarterOn]_/1(In1)
  Mode_StartButtonState[1Stim|2SoftECU]/1 -> Mode_StartButtonState[1Stim|2SoftECU]_/1(In1)
  Mode_Transmission[1Manual|2Automatic]_/1(Out1) -> Bus Creator/10  "Mode_Transmission[1Manual|2Automatic]"
  Sw_CrankShaft_Reset[0Disabled|1Enabled]_/1(Out1) -> Bus Creator/11  "Sw_CrankShaft_Reset[0Disabled|1Enabled]"
  Mode_Transmission[1Manual|2Automatic]/1 -> Mode_Transmission[1Manual|2Automatic]_/1(In1)
  Mode_StartButtonState[1Stim|2SoftECU]_/1(Out1) -> Bus Creator/12  "Mode_StartButtonState[1Stim|2SoftECU]"
  Sw_CrankShaft_Reset[0Disabled|1Enabled]/1 -> Sw_CrankShaft_Reset[0Disabled|1Enabled]_/1(In1)

== system ASM_Traffic_new/DomainControl/StartSystem/Interface_Out/Control_ModelSignals ==
  State_StartButton[-2|-1|0|1|2|3] : Inport
  Sw_Ignition[0|1] : Inport  Port=2
  Sw_StarterReq[0|1] : Inport  Port=3
  Bus Creator4 : BusCreator  Inputs=3
  State_StartButton[-2|-1|0|1|2|3]_ : Subsystem
      mask Display: disp('')
  Sw_Ignition[0|1]_ : Subsystem
      mask Display: disp('')
  Sw_StarterReq[0|1]_ : Subsystem
      mask Display: disp('')
  Out : Outport  VectorParamsAs1DForOutWhenUnconnected=off
  wires:
  Sw_StarterReq[0|1]_/1(Out1) -> Bus Creator4/3  "Sw_StarterReq[0|1]"
  Sw_Ignition[0|1]_/1(Out1) -> Bus Creator4/2  "Sw_Ignition[0|1]"
  Bus Creator4/1 -> Out/1  "Control"
  Sw_StarterReq[0|1]/1 -> Sw_StarterReq[0|1]_/1(In1)
  Sw_Ignition[0|1]/1 -> Sw_Ignition[0|1]_/1(In1)
  State_StartButton[-2|-1|0|1|2|3]/1 -> State_StartButton[-2|-1|0|1|2|3]_/1(In1)
  State_StartButton[-2|-1|0|1|2|3]_/1(Out1) -> Bus Creator4/1  "State_StartButton[-2|-1|0|1|2|3]"

== system ASM_Traffic_new/DomainControl/StartSystem/SignalInterface/ASMSignalInterface ==
  ASMSignalBus : Inport
  Enable : EnablePort
  signal_structure : Subsystem
  wires:
  ASMSignalBus/1 -> signal_structure/1(ASMSignalBus)

== system ASM_Traffic_new/DomainControl/StartSystem/SignalInterface/ExternalOutports ==
  In1 : Inport
  Enable : EnablePort
  Select_Outport_Signals : Subsystem
  StartSystem : dsmpblib/Data Outport  Tag=ASM_MPB  Priority=-10000
      settings: SourceProductName=dSPACE Model Interface Package for Simulink (MIPS)
  wires:
  In1/1 -> Select_Outport_Signals/1(ASMSignalBus)
  Select_Outport_Signals/6(State_StartButton[-2|-1|0|1|2|3]) -> StartSystem/6
  Select_Outport_Signals/5(Sw_StarterReq[0|1]) -> StartSystem/5
  Select_Outport_Signals/4(Sw_Ignition[0|1]) -> StartSystem/4
  Select_Outport_Signals/3(Sw_Acc[0|1]) -> StartSystem/3
  Select_Outport_Signals/2(Lock[0|1]) -> StartSystem/2
  Select_Outport_Signals/1(Flag_NotPressed_Pedal[0|1]) -> StartSystem/1

== system ASM_Traffic_new/DomainControl/TorqueManager/Control/SoftECU_TorqueManager ==
  UserInterface : Inport
  Interface_In : Inport  Port=2
  Bus Creator : BusCreator  Inputs=1
  Bus Creator7 : BusCreator  Inputs=5
  Bus Selector : BusSelector  OutputSignals=ExternalModel.Sw_Ignition[0|1],ExternalModel.Sw_StarterReq[0|1],ExternalModel.Pos_BrakePedal[%],ExternalModel.Sw_Starter[0Off|1On],ExternalModel.State_Engine[0|1|2|3|4]
  Terminator : Terminator
  ASMSignalBus : Outport  VectorParamsAs1DForOutWhenUnconnected=off
  Out : Outport  Port=2  VectorParamsAs1DForOutWhenUnconnected=off
  wires:
  Bus Creator7/1 -> Bus Creator/1  "ExternalModel"
  Bus Selector/4 -> Bus Creator7/4  "<Sw_Starter[0Off|1On]>"
  Bus Selector/3 -> Bus Creator7/3  "<Pos_BrakePedal[%]>"
  Bus Selector/2 -> Bus Creator7/2  "<Sw_StarterReq[0|1]>"
  Bus Selector/5 -> Bus Creator7/5  "<State_Engine[0|1|2|3|4]>"
  Bus Selector/1 -> Bus Creator7/1  "<Sw_Ignition[0|1]>"
  Interface_In/1 -> Bus Selector/1
  Bus Creator/1 -> Out/1, ASMSignalBus/1  "Control"
  UserInterface/1 -> Terminator/1

== system ASM_Traffic_new/DomainControl/TorqueManager/Control/UserInterface ==
  note: Torque Manager Basic
  In : Inport
  ASMSignalBus_Control : Subsystem
  DISP_Control : Subsystem
  PAR_Control : Subsystem
  Out : Outport  VectorParamsAs1DForOutWhenUnconnected=off
  wires:
  PAR_Control/1(Out) -> Out/1
  In/1 -> DISP_Control/1(In), ASMSignalBus_Control/1(In)

== system ASM_Traffic_new/DomainControl/TorqueManager/Interface_In/ModelSignals ==
  Sw_ModelPortBlocks[0Disabled|1Enabled] : Inport
  Sw_ModelDeskPlottingInterface[0Disabled|1Enabled] : Inport  Port=2
  Pos_BrakePedal[%] : Inport  Port=3
  State_Engine[0|1|2|3|4] : Inport  Port=4
  Sw_Ignition[0|1] : Inport  Port=5
  Sw_StarterReq[0|1] : Inport  Port=6
  Sw_Starter[0Off|1On] : Inport  Port=7
  Bus Creator : BusCreator  Inputs=7
  Pos_BrakePedal[%]_ : Subsystem
      mask Display: disp('')
  State_Engine[0|1|2|3|4]_ : Subsystem
      mask Display: disp('')
  Sw_Ignition[0|1]_ : Subsystem
      mask Display: disp('')
  Sw_ModelDeskPlottingInterface[0Disabled|1Enabled]_ : Subsystem
  Sw_ModelPortBlocks[0Disabled|1Enabled]_ : Subsystem
  Sw_StarterReq[0|1]_ : Subsystem
      mask Display: disp('')
  Sw_Starter[0Off|1On]_ : Subsystem
      mask Display: disp('')
  Out : Outport  VectorParamsAs1DForOutWhenUnconnected=off
  wires:
  Sw_ModelDeskPlottingInterface[0Disabled|1Enabled]_/1(Out1) -> Bus Creator/2  "Sw_ModelDeskPlottingInterface[0Disabled|1Enabled]"
  Sw_ModelPortBlocks[0Disabled|1Enabled]_/1(Out1) -> Bus Creator/1  "Sw_ModelPortBlocks[0Disabled|1Enabled]"
  Sw_ModelDeskPlottingInterface[0Disabled|1Enabled]/1 -> Sw_ModelDeskPlottingInterface[0Disabled|1Enabled]_/1(In1)
  Sw_ModelPortBlocks[0Disabled|1Enabled]/1 -> Sw_ModelPortBlocks[0Disabled|1Enabled]_/1(In1)
  Bus Creator/1 -> Out/1  "ExternalModel"
  State_Engine[0|1|2|3|4]_/1(Out1) -> Bus Creator/4  "State_Engine[0|1|2|3|4]"
  State_Engine[0|1|2|3|4]/1 -> State_Engine[0|1|2|3|4]_/1(In1)
  Pos_BrakePedal[%]/1 -> Pos_BrakePedal[%]_/1(In1)
  Pos_BrakePedal[%]_/1(Out1) -> Bus Creator/3  "Pos_BrakePedal[%]"
  Sw_Starter[0Off|1On]_/1(Out1) -> Bus Creator/7  "Sw_Starter[0Off|1On]"
  Sw_StarterReq[0|1]_/1(Out1) -> Bus Creator/6  "Sw_StarterReq[0|1]"
  Sw_StarterReq[0|1]/1 -> Sw_StarterReq[0|1]_/1(In1)
  Sw_Ignition[0|1]_/1(Out1) -> Bus Creator/5  "Sw_Ignition[0|1]"
  Sw_Starter[0Off|1On]/1 -> Sw_Starter[0Off|1On]_/1(In1)
  Sw_Ignition[0|1]/1 -> Sw_Ignition[0|1]_/1(In1)

== system ASM_Traffic_new/DomainControl/TorqueManager/Interface_Out/Control_ModelSignals ==
  Ignition_ICE[0Off|1On] : Inport
  StarterReq_ICE[0Off|1On] : Inport  Port=2
  Pos_BrakePedal_Desired[%] : Inport  Port=3
  Starter_Drivetrain[0Off|1On] : Inport  Port=4
  State_Engine[0|1|2|3|4] : Inport  Port=5
  " Mode_BSG[-1|0|1|2|3|4|5]" : Inport  Port=6
  Trq_Request_EM[Nm] : Inport  Port=7
  Trq_Request_ICE[Nm] : Inport  Port=8
  HybridMode_ICE[0Off|1OnIdle|2OnPower|3err] : Inport  Port=9
  Trq_Request_Brake[Nm] : Inport  Port=10
  Sw_DriveMode[0Hybrid|1ICE|2EM] : Inport  Port=11
  Vehicle_Topology[-2|-1|0|2] : Inport  Port=12
  " Mode_BSG[-1|0|1|2|3|4|5]_" : Subsystem
      mask Display: disp('')
  Bus Creator7 : BusCreator  Inputs=12
  HybridMode_ICE[0Off|1OnIdle|2OnPower|3err]_ : Subsystem
      mask Display: disp('')
  Ignition_ICE[0Off|1On]_ : Subsystem
      mask Display: disp('')
  Pos_BrakePedal_Desired[%]_ : Subsystem
      mask Display: disp('')
  StarterReq_ICE[0Off|1On]_ : Subsystem
      mask Display: disp('')
  Starter_Drivetrain[0Off|1On]_ : Subsystem
      mask Display: disp('')
  State_Engine[0|1|2|3|4]_ : Subsystem
      mask Display: disp('')
  Sw_DriveMode[0Hybrid|1ICE|2EM]_ : Subsystem
      mask Display: disp('')
  Trq_Request_Brake[Nm]_ : Subsystem
      mask Display: disp('')
  Trq_Request_EM[Nm]_ : Subsystem
      mask Display: disp('')
  Trq_Request_ICE[Nm]_ : Subsystem
      mask Display: disp('')
  Vehicle_Topology[-2|-1|0|2]_ : Subsystem
      mask Display: disp('')
  Out : Outport  VectorParamsAs1DForOutWhenUnconnected=off
  wires:
  Bus Creator7/1 -> Out/1  "Control"
  Ignition_ICE[0Off|1On]/1 -> Ignition_ICE[0Off|1On]_/1(In1)
  StarterReq_ICE[0Off|1On]_/1(Out1) -> Bus Creator7/2  "StarterReq_ICE[0Off|1On]"
  StarterReq_ICE[0Off|1On]/1 -> StarterReq_ICE[0Off|1On]_/1(In1)
  Ignition_ICE[0Off|1On]_/1(Out1) -> Bus Creator7/1  "Ignition_ICE[0Off|1On]"
  Pos_BrakePedal_Desired[%]/1 -> Pos_BrakePedal_Desired[%]_/1(In1)
  Pos_BrakePedal_Desired[%]_/1(Out1) -> Bus Creator7/3  "Pos_BrakePedal_Desired[%]"
  HybridMode_ICE[0Off|1OnIdle|2OnPower|3err]_/1(Out1) -> Bus Creator7/9  "HybridMode_ICE[0Off|1OnIdle|2OnPower|3err]"
  HybridMode_ICE[0Off|1OnIdle|2OnPower|3err]/1 -> HybridMode_ICE[0Off|1OnIdle|2OnPower|3err]_/1(In1)
  Trq_Request_ICE[Nm]_/1(Out1) -> Bus Creator7/8  "Trq_Request_ICE[Nm]"
  Trq_Request_ICE[Nm]/1 -> Trq_Request_ICE[Nm]_/1(In1)
  " Mode_BSG[-1|0|1|2|3|4|5]"/1 -> " Mode_BSG[-1|0|1|2|3|4|5]_"/1(In1)
  " Mode_BSG[-1|0|1|2|3|4|5]_"/1(Out1) -> Bus Creator7/6  "Mode_BSG[-1|0|1|2|3|4|5]"
  Trq_Request_EM[Nm]/1 -> Trq_Request_EM[Nm]_/1(In1)
  Trq_Request_EM[Nm]_/1(Out1) -> Bus Creator7/7  "Trq_Request_EM[Nm]"
  Starter_Drivetrain[0Off|1On]/1 -> Starter_Drivetrain[0Off|1On]_/1(In1)
  Starter_Drivetrain[0Off|1On]_/1(Out1) -> Bus Creator7/4  "Starter_Drivetrain[0Off|1On]"
  Trq_Request_Brake[Nm]_/1(Out1) -> Bus Creator7/10  "Trq_Request_Brake[Nm]"
  Trq_Request_Brake[Nm]/1 -> Trq_Request_Brake[Nm]_/1(In1)
  Sw_DriveMode[0Hybrid|1ICE|2EM]/1 -> Sw_DriveMode[0Hybrid|1ICE|2EM]_/1(In1)
  Sw_DriveMode[0Hybrid|1ICE|2EM]_/1(Out1) -> Bus Creator7/11  "Sw_DriveMode[0Hybrid|1ICE|2EM]"
  State_Engine[0|1|2|3|4]/1 -> State_Engine[0|1|2|3|4]_/1(In1)
  State_Engine[0|1|2|3|4]_/1(Out1) -> Bus Creator7/5  "State_Engine[0|1|2|3|4]"
  Vehicle_Topology[-2|-1|0|2]_/1(Out1) -> Bus Creator7/12  "Vehicle_Topology[-2|-1|0|2]"
  Vehicle_Topology[-2|-1|0|2]/1 -> Vehicle_Topology[-2|-1|0|2]_/1(In1)

== system ASM_Traffic_new/DomainControl/TorqueManager/SignalInterface/ASMSignalInterface ==
  ASMSignalBus : Inport
  Enable : EnablePort
  signal_structure : Subsystem
  wires:
  ASMSignalBus/1 -> signal_structure/1(ASMSignalBus)

== system ASM_Traffic_new/DomainControl/TorqueManager/SignalInterface/ExternalOutports ==
  In1 : Inport
  Enable : EnablePort
  Select_Outport_Signals : Subsystem
  TorqueManager : dsmpblib/Data Outport  Tag=ASM_MPB  Priority=-10000
      settings: SourceProductName=dSPACE Model Interface Package for Simulink (MIPS)
  wires:
  In1/1 -> Select_Outport_Signals/1(ASMSignalBus)
  Select_Outport_Signals/5(Sw_Starter[0Off|1On]) -> TorqueManager/5
  Select_Outport_Signals/4(Sw_StarterReq[0|1]) -> TorqueManager/4
  Select_Outport_Signals/3(State_Engine[0|1|2|3|4]) -> TorqueManager/3
  Select_Outport_Signals/2(Pos_BrakePedal[%]) -> TorqueManager/2
  Select_Outport_Signals/1(Sw_Ignition[0|1]) -> TorqueManager/1

== system ASM_Traffic_new/Driver/Interface_In/ModelSignals/Angle_SteeringWheel_Maneuver[deg]_ ==
  In1 : Inport
  DummyGain : Gain  SaturateOnIntegerOverflow=on  OutDataTypeStr=Inherit: Same as input  ParamDataTypeStr=Inherit: Same as input
  Out1 : Outport  VectorParamsAs1DForOutWhenUnconnected=off
  wires:
  DummyGain/1 -> Out1/1
  In1/1 -> DummyGain/1

== system ASM_Traffic_new/Driver/Interface_In/ModelSignals/Angle_Yaw_Veh_Road[deg]_ ==
  In1 : Inport
  Gain : Gain  SaturateOnIntegerOverflow=on  OutDataTypeStr=Inherit: Same as input  ParamDataTypeStr=Inherit: Same as input
  Out1 : Outport  VectorParamsAs1DForOutWhenUnconnected=off
  wires:
  In1/1 -> Gain/1
  Gain/1 -> Out1/1

== system ASM_Traffic_new/Driver/Interface_In/ModelSignals/Angle_Yaw_Vehicle_CoorSys_E[deg]_ ==
  In1 : Inport
  DummyGain : Gain  SaturateOnIntegerOverflow=on  OutDataTypeStr=Inherit: Same as input  ParamDataTypeStr=Inherit: Same as input
  Out1 : Outport  VectorParamsAs1DForOutWhenUnconnected=off
  wires:
  DummyGain/1 -> Out1/1
  In1/1 -> DummyGain/1

== system ASM_Traffic_new/Driver/Interface_In/ModelSignals/CorneringStiffness_Tire_Front[N|rad]_ ==
  In1 : Inport
  DummyGain : Gain  SaturateOnIntegerOverflow=on  OutDataTypeStr=Inherit: Same as input  ParamDataTypeStr=Inherit: Same as input
  Out1 : Outport  VectorParamsAs1DForOutWhenUnconnected=off
  wires:
  DummyGain/1 -> Out1/1
  In1/1 -> DummyGain/1

== system ASM_Traffic_new/Driver/Interface_In/ModelSignals/CorneringStiffness_Tire_Rear[N|rad]_ ==
  In1 : Inport
  DummyGain : Gain  SaturateOnIntegerOverflow=on  OutDataTypeStr=Inherit: Same as input  ParamDataTypeStr=Inherit: Same as input
  Out1 : Outport  VectorParamsAs1DForOutWhenUnconnected=off
  wires:
  In1/1 -> DummyGain/1
  DummyGain/1 -> Out1/1

== system ASM_Traffic_new/Driver/Interface_In/ModelSignals/Curv_Preview_Road[1|m]_ ==
  In1 : Inport
  Gain : Gain  SaturateOnIntegerOverflow=on  OutDataTypeStr=Inherit: Same as input  ParamDataTypeStr=Inherit: Same as input
  Out1 : Outport  VectorParamsAs1DForOutWhenUnconnected=off
  wires:
  Gain/1 -> Out1/1
  In1/1 -> Gain/1

== system ASM_Traffic_new/Driver/Interface_In/ModelSignals/Curv_Veh_Road[1|m]_ ==
  In1 : Inport
  Gain : Gain  SaturateOnIntegerOverflow=on  OutDataTypeStr=Inherit: Same as input  ParamDataTypeStr=Inherit: Same as input
  Out1 : Outport  VectorParamsAs1DForOutWhenUnconnected=off
  wires:
  Gain/1 -> Out1/1
  In1/1 -> Gain/1

== system ASM_Traffic_new/Driver/Interface_In/ModelSignals/Dist_Border_Left[m]_ ==
  In1 : Inport
  Gain : Gain  SaturateOnIntegerOverflow=on  OutDataTypeStr=Inherit: Same as input  ParamDataTypeStr=Inherit: Same as input
  Out1 : Outport  VectorParamsAs1DForOutWhenUnconnected=off
  wires:
  Gain/1 -> Out1/1
  In1/1 -> Gain/1

== system ASM_Traffic_new/Driver/Interface_In/ModelSignals/Dist_Border_Right[m]_ ==
  In1 : Inport
  Gain : Gain  SaturateOnIntegerOverflow=on  OutDataTypeStr=Inherit: Same as input  ParamDataTypeStr=Inherit: Same as input
  Out1 : Outport  VectorParamsAs1DForOutWhenUnconnected=off
  wires:
  In1/1 -> Gain/1
  Gain/1 -> Out1/1

== system ASM_Traffic_new/Driver/Interface_In/ModelSignals/Enable_v_Init[0|1]_ ==
  In1 : Inport
  DummyGain : Gain  SaturateOnIntegerOverflow=on  OutDataTypeStr=Inherit: Same as input  ParamDataTypeStr=Inherit: Same as input
  Out1 : Outport  VectorParamsAs1DForOutWhenUnconnected=off
  wires:
  In1/1 -> DummyGain/1
  DummyGain/1 -> Out1/1

== system ASM_Traffic_new/Driver/Interface_In/ModelSignals/F_Driving_Res[N]_ ==
  In1 : Inport
  DummyGain : Gain  SaturateOnIntegerOverflow=on  OutDataTypeStr=Inherit: Same as input  ParamDataTypeStr=Inherit: Same as input
  Out1 : Outport  VectorParamsAs1DForOutWhenUnconnected=off
  wires:
  In1/1 -> DummyGain/1
  DummyGain/1 -> Out1/1

== system ASM_Traffic_new/Driver/Interface_In/ModelSignals/Gear_Maneuver[]_ ==
  In1 : Inport
  DummyGain : Gain  SaturateOnIntegerOverflow=on  OutDataTypeStr=Inherit: Same as input  ParamDataTypeStr=Inherit: Same as input
  Out1 : Outport  VectorParamsAs1DForOutWhenUnconnected=off
  wires:
  In1/1 -> DummyGain/1
  DummyGain/1 -> Out1/1

== system ASM_Traffic_new/Driver/Interface_In/ModelSignals/Gear_Max[0Off|1_n]_ ==
  In1 : Inport
  DummyGain : Gain  SaturateOnIntegerOverflow=on  OutDataTypeStr=Inherit: Same as input  ParamDataTypeStr=Inherit: Same as input
  Out1 : Outport  VectorParamsAs1DForOutWhenUnconnected=off
  wires:
  In1/1 -> DummyGain/1
  DummyGain/1 -> Out1/1

== system ASM_Traffic_new/Driver/Interface_In/ModelSignals/Inertia_z_Vehicle_Total[kgm2]_ ==
  In1 : Inport
  DummyGain : Gain  SaturateOnIntegerOverflow=on  OutDataTypeStr=Inherit: Same as input  ParamDataTypeStr=Inherit: Same as input
  Out1 : Outport  VectorParamsAs1DForOutWhenUnconnected=off
  wires:
  In1/1 -> DummyGain/1
  DummyGain/1 -> Out1/1

== system ASM_Traffic_new/Driver/Interface_In/ModelSignals/Lane_ID_Vehicle[]_ ==
  In1 : Inport
  DummyGain : Gain  SaturateOnIntegerOverflow=on  OutDataTypeStr=Inherit: Same as input  ParamDataTypeStr=Inherit: Same as input
  Out1 : Outport  VectorParamsAs1DForOutWhenUnconnected=off
  wires:
  In1/1 -> DummyGain/1
  DummyGain/1 -> Out1/1
